simulink model "EV6_LUT_FourWheel_EV6Battery77p4kWh_PowerCorrected"  (R2024a)
settings: Solver=ode4  StartTime=0  StopTime=60  FixedStep=0.001  RelTol=1e-3
PreLoadFcn:
  | VSS_BICYCLE=Simulink.Variant('Dual=0');
  | VSS_DUAL=Simulink.Variant('Dual=1');
  | Dual=1;
  | load('DriveCycle2.mat')
PostLoadFcn:
  | if any(exist('dsrtsu_mdlpostloadfcn', 'file') ~= 0), dsrtsu_mdlpostloadfcn('Execute', bdroot); end
InitFcn:
  | , if any(exist('rtifpga_mdlclblib', 'file') ~= 0), rtifpga_mdlclblib('Init', bdroot); end,
  | , if any(exist('dsmpb_private', 'file') ~= 0), dsmpb_private('dsmpb_mdlclblib', 'Init', bdroot); end,
  | load('DriveCycle2.mat')
model workspace (MAT data in the model file):
  DiffRatio = 10.65
  EV6_2023_BattBranchCapacity_Ah = 55.5236728838
  EV6_2023_BattEnergy_kWh = 77.4
  EV6_2023_BattNominalVoltage_V = 697
  EV6_2023_BattNumCellsParallel = 2
  EV6_2023_BattNumCellsSeries = 192
  EV6_2023_BattOpenVoltCapBpts = [0 0.1 0.2 0.3 0.4 0.5 0.6 0.7 0.8 0.9 1]
  EV6_2023_BattOpenVoltTbl = [2.96762142548 3.40364281191 3.47417488548 3.54470541822 3.61523441014 3.68576186124 3.75628777151 3.82681214095 3.94527005036 4.07101207308 4.2120755254]
  EV6_2023_BattPackCapacity_Ah = 111.047345768
  EV6_2023_BattResistSocBpts = [0 0.2 0.4 0.6 0.8 1]
  EV6_2023_BattResistTbl = [0.0163620057716 0.0118174152018 0.00807187352333 0.00375663957972 0.00266904525531 0.00103635901355 0.0019014404175 0.0172368903217 0.0121226074867 0.00758541551769 0.00474065349228 0.00337561163613 ... (42 elements, 7x6)]
  EV6_2023_BattResistTempBpts = [243.1 253.1 263.1 273.1 283.1 298.1 313.1]
  EV6_2023_InitialPackOCV_V = 726.471714233
  EV6_2023_InitialSOC = 0.638878863672
  EV6_BattCellCapacity_Ah = 60.3
  EV6_BattInitialSOC = 0.638878863672
  EV6_BattOCV_Cell_V = [2.96762142548 3.40364281191 3.47417488548 3.54470541822 3.61523441014 3.68576186124 3.75628777151 3.82681214095 3.94527005036 4.07101207308 4.2120755254]
  EV6_BattOCV_SOC = [0 0.1 0.2 0.3 0.4 0.5 0.6 0.7 0.8 0.9 1]
  EV6_BattPackCapacity_Ah = 120.6
  EV6_BattParallelCells = 2
  EV6_BattResistanceSOC = [0 0.2 0.4 0.6 0.8 1]
  EV6_BattResistanceTable_Ohm = [0.0163620057716 0.0118174152018 0.00807187352333 0.00375663957972 0.00266904525531 0.00103635901355 0.0019014404175 0.0172368903217 0.0121226074867 0.00758541551769 0.00474065349228 0.00337561163613 ... (42 elements, 7x6)]
  EV6_BattResistanceTemp_K = [243.1 253.1 263.1 273.1 283.1 298.1 313.1]
  EV6_BattSeriesCells = 192
  EV6_FinalDriveRatio = 10.65
  EV6_TargetPackResistance_Ohm = 0.132763804608
  Gas = 0.383333333333
undefined symbols (not defined in the file): accel_bp_mps2, AccelCmd, ActTqLF_Nm_, ActTqLR_Nm_, ActTqRF_Nm_, ActTqRR_Nm_, BattChargeLimitMaxPwr, BattChargeLimitSocBpts, BattChargeLimitTbl, BattDischargeLimitSocBpts, BattDischargeLimitTbl, BattDischargeMaxPwr, BrakeMaxPrs, BrakeMaxTrq, ChassisDistCg2FrontAxle, ChassisDistCg2RearAxle, ChassisVehMass, CltchCmd, CoastDown, DecelCmd, DiscIntNeverNeededParam, EnvGravCnst, EnvPrs, EnvTemp, EV6_RegenTorqueGain, EV6_TractionTorqueGain, front_share_regen_3d, front_share_traction_3d, FuelSpecificGrav, GearCmd, h, InitStates, lgSw, limitedMCT, MCT, MtrEffSpdBpts, MtrEffTbl, MtrEffTrqBpts, MtrPwrMax, MtrTrqMax, out_1, pMCT, RealSimPara, Ref_speed, Ref_time, regen_torque_bp_Nm, speed_bp_kph, SteeringCmd, SupvsryCtrlRegenBrkCutOffTbl, SupvsryCtrlRegenSpdBpts, TestScnrioCycleNum, traction_torque_bp_Nm, US06, VEH
libraries: VSIGenLib x65, simulink x54, etargetslib x38, dsmpblib x24, vehdynlibtire x12, autolibshared x11, vehdynlibsuspension x7, vehdynlibtirecommon x7, autolibpowerinfoutils x6, autolibutils x5, autolibsharedcoupling x4, autolibmappedmotor x4
(part 8 of 19)

== system EV6_LUT_FourWheel_EV6Battery77p4kWh_PowerCorrected/Vehicle Under Test1/Vehicle/Powertrain Supervisory Controller /Engine Torque Command/EV6 Torque Distribution ==
  Accel_mps2 : Inport
  Speed_kph : Inport  Port=2
  MtrTrqCmd : Inport  Port=3
  Regen Brake Split LUT : Subsystem
  Select Front Share : Switch  SaturateOnIntegerOverflow=off  InputSameDT=off
  Select Front Torque : Switch  SaturateOnIntegerOverflow=off  InputSameDT=off
  Select Rear Share : Switch  SaturateOnIntegerOverflow=off  InputSameDT=off
  Select Rear Torque : Switch  SaturateOnIntegerOverflow=off  InputSameDT=off
  Share Sum : Sum
  Share Sum Display : Display
  Torque Error : Sum  Inputs=+-
  Torque Error Display : Display
  Torque Sum : Sum
  Traction Torque Split LUT : Subsystem
  FrontShare : Outport
  RearShare : Outport  Port=2
  FrontMtrTrqCmd : Outport  Port=3
  RearMtrTrqCmd : Outport  Port=4
  wires:
  Accel_mps2/1 -> Traction Torque Split LUT/1(Accel_mps2), Regen Brake Split LUT/1(Accel_mps2)
  Speed_kph/1 -> Traction Torque Split LUT/2(Speed_kph), Regen Brake Split LUT/2(Speed_kph)
  MtrTrqCmd/1 -> Select Rear Torque/2, Torque Error/2, Select Front Torque/2, Select Front Share/2, Select Rear Share/2, Traction Torque Split LUT/3(MtrTrqCmd), Regen Brake Split LUT/3(MtrTrqCmd)
  Traction Torque Split LUT/1(FrontShare) -> Select Front Share/1
  Regen Brake Split LUT/1(FrontShare) -> Select Front Share/3
  Traction Torque Split LUT/2(RearShare) -> Select Rear Share/1
  Regen Brake Split LUT/2(RearShare) -> Select Rear Share/3
  Traction Torque Split LUT/3(FrontMtrTrqCmd) -> Select Front Torque/1
  Regen Brake Split LUT/3(FrontMtrTrqCmd) -> Select Front Torque/3
  Traction Torque Split LUT/4(RearMtrTrqCmd) -> Select Rear Torque/1
  Regen Brake Split LUT/4(RearMtrTrqCmd) -> Select Rear Torque/3
  Select Front Share/1 -> FrontShare/1, Share Sum/1
  Select Rear Share/1 -> RearShare/1, Share Sum/2
  Select Front Torque/1 -> FrontMtrTrqCmd/1, Torque Sum/1
  Select Rear Torque/1 -> RearMtrTrqCmd/1, Torque Sum/2
  Share Sum/1 -> Share Sum Display/1
  Torque Sum/1 -> Torque Error/1
  Torque Error/1 -> Torque Error Display/1

== system EV6_LUT_FourWheel_EV6Battery77p4kWh_PowerCorrected/Vehicle Under Test1/Vehicle/Powertrain Supervisory Controller /Engine Torque Command/Motor Torque Arbitration and Power Management ==
  MotTrqCmdTrac : Inport
  AccelPdl : Inport  Port=2
  BattPwrDisChrgLmt : Inport  Port=3
  "BattPwrChrgLmt " : Inport  Port=4
  MotSpd : Inport  Port=5
  MotTrqCmdRegen : Inport  Port=6
  Accel Decel Switch : Switch  Criteria=u2 > Threshold  SaturateOnIntegerOverflow=off  InputSameDT=off
  Compare To Constant : simulink/Logic and Bit Operations/Compare To Constant  relop=>  const=0  OutDataTypeStr=boolean
  Power Management : Subsystem
  MotTrqCmdFinal : Outport  VectorParamsAs1DForOutWhenUnconnected=off
  wires:
  AccelPdl/1 -> Compare To Constant/1
  MotTrqCmdRegen/1 -> Accel Decel Switch/3
  MotTrqCmdTrac/1 -> Accel Decel Switch/1
  Power Management/1(MotTrqCmdFinal) -> MotTrqCmdFinal/1
  Accel Decel Switch/1 -> Power Management/4(MotTrqCmd)
  BattPwrDisChrgLmt/1 -> Power Management/1(BattPwrDischrgLmt)
  "BattPwrChrgLmt "/1 -> Power Management/2(BattPwrChrgLmt)
  MotSpd/1 -> Power Management/3(MotSpd)
  Compare To Constant/1 -> Accel Decel Switch/2

== system EV6_LUT_FourWheel_EV6Battery77p4kWh_PowerCorrected/Vehicle Under Test1/Vehicle/Powertrain Supervisory Controller /Engine Torque Command/Series Regen Braking ==
  note: - Total brake torque request based on brake pressure and parameters of disc brakes
      | - Use as much regenerative motor braking as possible
      | - Any braking torque request that cannot be provided by the motor, will be provided by the friction brakes
  note: These are all torque on wheels, which is DiffRatio*torque on motor
  BattSoc : Inport
  VehSpd : Inport  Port=2
  MotSpd : Inport  Port=3
  "DecelCmd " : Inport  Port=4
  BrkTrqReqTotal Display : Display
  ChrgLmt : Lookup_n-D  NumberOfTableDimensions=1  BreakpointsForDimension1=BattChargeLimitSocBpts  Table=BattChargeLimitTbl  ExtrapMethod=Clip  UseLastTableValue=on  InternalRulePriority=Speed  RndMeth=Simplest
  ChrgLmt Display : Display
  DecelCmd input : Display
  Display : Display
  Gain : Gain  Gain=-1
  Gain1 : Gain  Gain=BrakeMaxTrq
  Gain2 : Gain  Gain=1/BrakeMaxTrq
  Gain3 : Gain  Gain=EV6_FinalDriveRatio
  Max Motor Torque : LibPtSupervisoryCtrl/Powertrain Supervisory Controller /Engine Torque Command/Accel Pedal to Traction Wheel Torque Request/Max Motor Torque  SystemSampleTime=-1  VariantActivationTime=update diagram  AllowFlexibleInterface=on  Latency=0  AutoFrameSizeCalculation=off
  MinMax : MinMax  Inputs=2
  MotSpd Display : Display
  MotTrqCmdRegen : Display
  MotTrqReflectedToWheels1 : Gain  Commented=on  Gain=DiffRatio
  Product1 : Product
  Product3 : Product
  RegenBraking Display : Display
  RegenBrakingCutoff : Lookup_n-D  NumberOfTableDimensions=1  BreakpointsForDimension1=SupvsryCtrlRegenSpdBpts  Table=SupvsryCtrlRegenBrkCutOffTbl  ExtrapMethod=Clip  UseLastTableValue=on  InternalRulePriority=Speed  RndMeth=Simplest
  RegenFactor Display : Display
  Saturation : Saturate  UpperLimit=1  LowerLimit=0
  Saturation1 : Saturate  UpperLimit=1  LowerLimit=0
  Scope{,1..6} (7 alike) : Scope
  Subtract : Sum  Inputs=+-
  VehSpd Display : Display
  WhlTrqReflectedToMot : Gain  Gain=1/EV6_FinalDriveRatio
  WhlTrqReflectedToMot1 : Gain  Commented=on  Gain=1/DiffRatio
  " MotTrqCmdRegen" : Outport  VectorParamsAs1DForOutWhenUnconnected=off
  " BrkCmd" : Outport  Port=2  VectorParamsAs1DForOutWhenUnconnected=off
  wires:
  Gain1/1 -> Scope/1, Subtract/1, MinMax/1  "BrkTrqReqTotal"
  Product3/1 -> WhlTrqReflectedToMot/1, Subtract/2  "MotTrqRegenWhl"
  Saturation1/1 -> Scope3/1, " BrkCmd"/1
  Max Motor Torque/1 -> Gain3/1, Scope6/1  "MotTrqMax"
  MinMax/1 -> Product3/1  "min"
  ChrgLmt/1 -> ChrgLmt Display/1, Product1/2
  VehSpd/1 -> VehSpd Display/1, RegenBrakingCutoff/1
  RegenBrakingCutoff/1 -> RegenBraking Display/1, Product1/1
  Product1/1 -> RegenFactor Display/1, Scope5/1, Product3/2  "RegenFactor"
  BattSoc/1 -> ChrgLmt/1
  MotSpd/1 -> MotSpd Display/1, Max Motor Torque/1
  Gain3/1 -> Scope1/1, MinMax/2  "MotTrqMaxWhls"
  WhlTrqReflectedToMot/1 -> Gain/1
  Gain/1 -> MotTrqCmdRegen/1, Scope4/1, " MotTrqCmdRegen"/1  "MotTrqCmdRegen"
  "DecelCmd "/1 -> Saturation/1, DecelCmd input/1  "BrkPrsReq"
  Saturation/1 -> Display/1, Scope2/1, Gain1/1
  Subtract/1 -> Gain2/1
  Gain2/1 -> BrkTrqReqTotal Display/1, Saturation1/1  "BrkTrqReqTotal"

== system EV6_LUT_FourWheel_EV6Battery77p4kWh_PowerCorrected/Vehicle Under Test1/Vehicle/Rear Wheel Drive/Ideal Diff/Power Bus ==
  DriveshftTrq : Inport
  Speed : Inport  Port=2
  Bus Creator : BusCreator  Inputs=1
  Bus Creator5 : BusCreator  Inputs=2
  Bus Creator6 : BusCreator  Inputs=3
  Bus Creator7 : BusCreator  Inputs=1
  Constant : Constant  Value=0
  Constant1 : Constant  Value=0
  Constant2 : Constant  Value=0
  Demux : Demux  Outputs=3
  Power Accounting Bus Creator : autolibpowerinfoutils/Power Accounting Bus Creator  AssctBlkSelPopup=Parent reference block  RefBlkName='autolibshareddiff/Open Differential'  PwrTrnsfrdCheckBox=on  PwrNotTrnsfrdCheckBox=on  PwrStoredCheckBox=on  aMode=aMode
  Signal Specification5 : SignalSpecification  Unit=W
  Transferred Power : Product
  Vector Concatenate : Concatenate  NumInputs=3
  PwrInfo : Outport
  wires:
  Constant2/1 -> Bus Creator7/1  "PwrStoredShft"
  Constant1/1 -> Bus Creator5/2  "PwrDampLoss"
  Vector Concatenate/1 -> Demux/1
  Speed/1 -> Transferred Power/2
  Demux/1 -> Bus Creator6/1  "PwrDriveshft"
  Demux/2 -> Bus Creator6/2  "PwrAxl1"
  Bus Creator7/1 -> Power Accounting Bus Creator/3
  DriveshftTrq/1 -> Transferred Power/1
  Demux/3 -> Bus Creator6/3  "PwrAxl2"
  Constant/1 -> Bus Creator5/1  "PwrMechLoss"
  Signal Specification5/1 -> Vector Concatenate/1, Vector Concatenate/2, Vector Concatenate/3  "PwrDriveshft"
  Transferred Power/1 -> Signal Specification5/1
  Bus Creator6/1 -> Bus Creator/1  "PwrTrnsfrd"
  Bus Creator5/1 -> Power Accounting Bus Creator/2
  Power Accounting Bus Creator/1 -> PwrInfo/1  "PwrInfo"
  Bus Creator/1 -> Power Accounting Bus Creator/1

== system EV6_LUT_FourWheel_EV6Battery77p4kWh_PowerCorrected/Vehicle Under Test1/Vehicle/Rear Wheel Drive/Ideal Diff AWD/Power Bus ==
  DriveshftTrq : Inport
  Speed : Inport  Port=2
  Bus Creator : BusCreator  Inputs=1
  Bus Creator5 : BusCreator  Inputs=2
  Bus Creator6 : BusCreator  Inputs=3
  Bus Creator7 : BusCreator  Inputs=1
  Constant : Constant  Value=0
  Constant1 : Constant  Value=0
  Constant2 : Constant  Value=0
  Demux : Demux  Outputs=3
  Power Accounting Bus Creator : autolibpowerinfoutils/Power Accounting Bus Creator  AssctBlkSelPopup=Parent reference block  RefBlkName='autolibshareddiff/Open Differential'  PwrTrnsfrdCheckBox=on  PwrNotTrnsfrdCheckBox=on  PwrStoredCheckBox=on  aMode=aMode
  Signal Specification5 : SignalSpecification  Unit=W
  Transferred Power : Product
  Vector Concatenate : Concatenate  NumInputs=3
  PwrInfo : Outport
  wires:
  Constant2/1 -> Bus Creator7/1  "PwrStoredShft"
  Constant1/1 -> Bus Creator5/2  "PwrDampLoss"
  Vector Concatenate/1 -> Demux/1
  Speed/1 -> Transferred Power/2
  Demux/1 -> Bus Creator6/1  "PwrDriveshft"
  Demux/2 -> Bus Creator6/2  "PwrAxl1"
  Bus Creator7/1 -> Power Accounting Bus Creator/3
  DriveshftTrq/1 -> Transferred Power/1
  Demux/3 -> Bus Creator6/3  "PwrAxl2"
  Constant/1 -> Bus Creator5/1  "PwrMechLoss"
  Signal Specification5/1 -> Vector Concatenate/1, Vector Concatenate/2, Vector Concatenate/3  "PwrDriveshft"
  Transferred Power/1 -> Signal Specification5/1
  Bus Creator6/1 -> Bus Creator/1  "PwrTrnsfrd"
  Bus Creator5/1 -> Power Accounting Bus Creator/2
  Power Accounting Bus Creator/1 -> PwrInfo/1  "PwrInfo"
  Bus Creator/1 -> Power Accounting Bus Creator/1

== system EV6_LUT_FourWheel_EV6Battery77p4kWh_PowerCorrected/Vehicle Under Test1/Vehicle/Rear Wheel Drive/Real Diff/Power Bus ==
  DriveshftTrq : Inport
  Speed : Inport  Port=2
  Bus Creator : BusCreator  Inputs=1
  Bus Creator5 : BusCreator  Inputs=2
  Bus Creator6 : BusCreator  Inputs=3
  Bus Creator7 : BusCreator  Inputs=1
  Constant : Constant  Value=0
  Constant1 : Constant  Value=0
  Constant2 : Constant  Value=0
  Demux : Demux  Outputs=3
  Power Accounting Bus Creator : autolibpowerinfoutils/Power Accounting Bus Creator  AssctBlkSelPopup=Parent reference block  RefBlkName='autolibshareddiff/Open Differential'  PwrTrnsfrdCheckBox=on  PwrNotTrnsfrdCheckBox=on  PwrStoredCheckBox=on  aMode=aMode
  Signal Specification5 : SignalSpecification  Unit=W
  Transferred Power : Product
  Vector Concatenate : Concatenate  NumInputs=3
  PwrInfo : Outport
  wires:
  Constant2/1 -> Bus Creator7/1  "PwrStoredShft"
  Constant1/1 -> Bus Creator5/2  "PwrDampLoss"
  Vector Concatenate/1 -> Demux/1
  Speed/1 -> Transferred Power/2
  Demux/1 -> Bus Creator6/1  "PwrDriveshft"
  Demux/2 -> Bus Creator6/2  "PwrAxl1"
  Bus Creator7/1 -> Power Accounting Bus Creator/3
  DriveshftTrq/1 -> Transferred Power/1
  Demux/3 -> Bus Creator6/3  "PwrAxl2"
  Constant/1 -> Bus Creator5/1  "PwrMechLoss"
  Signal Specification5/1 -> Vector Concatenate/1, Vector Concatenate/2, Vector Concatenate/3  "PwrDriveshft"
  Transferred Power/1 -> Signal Specification5/1
  Bus Creator6/1 -> Bus Creator/1  "PwrTrnsfrd"
  Bus Creator5/1 -> Power Accounting Bus Creator/2
  Power Accounting Bus Creator/1 -> PwrInfo/1  "PwrInfo"
  Bus Creator/1 -> Power Accounting Bus Creator/1

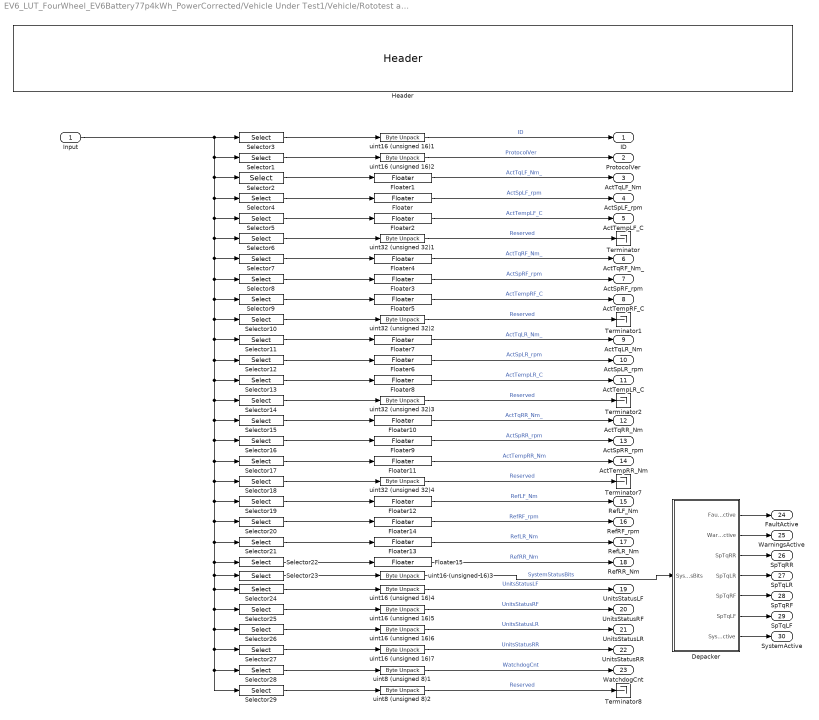
== system EV6_LUT_FourWheel_EV6Battery77p4kWh_PowerCorrected/Vehicle Under Test1/Vehicle/Rototest and ORNL Interface/From Rototest/RotoTestEthRX ==
  Input : Inport
  Depacker : Subsystem
  Floater{,1..15} (16 alike) : VSIGenLib/Floater  SystemSampleTime=-1  VariantActivationTime=update diagram  AllowFlexibleInterface=on  Latency=0  AutoFrameSizeCalculation=off
  Header : VSIGenLib/Header  not=''
  Selector1 : Selector  IndexMode=Zero-based  InputPortWidth=96  IndexOptions=Index vector (dialog)  Indices=[3 2]  OutputSizes=1
  Selector10 : Selector  IndexMode=Zero-based  InputPortWidth=96  IndexOptions=Index vector (dialog)  Indices=[35 34 33 32]  OutputSizes=1
  Selector11 : Selector  IndexMode=Zero-based  InputPortWidth=96  IndexOptions=Index vector (dialog)  Indices=[39 38 37 36]  OutputSizes=1
  Selector12 : Selector  IndexMode=Zero-based  InputPortWidth=96  IndexOptions=Index vector (dialog)  Indices=[43 42 41 40]  OutputSizes=1
  Selector13 : Selector  IndexMode=Zero-based  InputPortWidth=96  IndexOptions=Index vector (dialog)  Indices=[47 46 45 44]  OutputSizes=1
  Selector14 : Selector  IndexMode=Zero-based  InputPortWidth=96  IndexOptions=Index vector (dialog)  Indices=[51 50 49 48]  OutputSizes=1
  Selector15 : Selector  IndexMode=Zero-based  InputPortWidth=96  IndexOptions=Index vector (dialog)  Indices=[55 54 53 52]  OutputSizes=1
  Selector16 : Selector  IndexMode=Zero-based  InputPortWidth=96  IndexOptions=Index vector (dialog)  Indices=[59 58 57 56]  OutputSizes=1
  Selector17 : Selector  IndexMode=Zero-based  InputPortWidth=96  IndexOptions=Index vector (dialog)  Indices=[63 62 61 60]  OutputSizes=1
  Selector18 : Selector  IndexMode=Zero-based  InputPortWidth=96  IndexOptions=Index vector (dialog)  Indices=[67 66 65 64]  OutputSizes=1
  Selector19 : Selector  IndexMode=Zero-based  InputPortWidth=96  IndexOptions=Index vector (dialog)  Indices=[71 70 69 68]  OutputSizes=1
  Selector2 : Selector  IndexMode=Zero-based  InputPortWidth=96  IndexOptions=Index vector (dialog)  Indices=[7 6 5 4]  OutputSizes=1
  Selector20 : Selector  IndexMode=Zero-based  InputPortWidth=96  IndexOptions=Index vector (dialog)  Indices=[75 74 73 72]  OutputSizes=1
  Selector21 : Selector  IndexMode=Zero-based  InputPortWidth=96  IndexOptions=Index vector (dialog)  Indices=[79 78 77 76]  OutputSizes=1
  Selector22 : Selector  IndexMode=Zero-based  InputPortWidth=96  IndexOptions=Index vector (dialog)  Indices=[83 82 81 80]  OutputSizes=1
  Selector23 : Selector  IndexMode=Zero-based  InputPortWidth=96  IndexOptions=Index vector (dialog)  Indices=[85 84]  OutputSizes=1
  Selector24 : Selector  IndexMode=Zero-based  InputPortWidth=96  IndexOptions=Index vector (dialog)  Indices=[87 86]  OutputSizes=1
  Selector25 : Selector  IndexMode=Zero-based  InputPortWidth=96  IndexOptions=Index vector (dialog)  Indices=[89 88]  OutputSizes=1
  Selector26 : Selector  IndexMode=Zero-based  InputPortWidth=96  IndexOptions=Index vector (dialog)  Indices=[91 90]  OutputSizes=1
  Selector27 : Selector  IndexMode=Zero-based  InputPortWidth=96  IndexOptions=Index vector (dialog)  Indices=[93 92]  OutputSizes=1
  Selector28 : Selector  IndexMode=Zero-based  InputPortWidth=96  IndexOptions=Index vector (dialog)  Indices=[94]  OutputSizes=1
  Selector29 : Selector  IndexMode=Zero-based  InputPortWidth=96  IndexOptions=Index vector (dialog)  Indices=[95]  OutputSizes=1
  Selector3 : Selector  IndexMode=Zero-based  InputPortWidth=96  IndexOptions=Index vector (dialog)  Indices=[1 0]  OutputSizes=1
  Selector4 : Selector  IndexMode=Zero-based  InputPortWidth=96  IndexOptions=Index vector (dialog)  Indices=[11 10 9 8]  OutputSizes=1
  Selector5 : Selector  IndexMode=Zero-based  InputPortWidth=96  IndexOptions=Index vector (dialog)  Indices=[15 14 13 12]  OutputSizes=1
  Selector6 : Selector  IndexMode=Zero-based  InputPortWidth=96  IndexOptions=Index vector (dialog)  Indices=[19 18 17 16]  OutputSizes=1
  Selector7 : Selector  IndexMode=Zero-based  InputPortWidth=96  IndexOptions=Index vector (dialog)  Indices=[23 22 21 20]  OutputSizes=1
  Selector8 : Selector  IndexMode=Zero-based  InputPortWidth=96  IndexOptions=Index vector (dialog)  Indices=[27 26 25 24]  OutputSizes=1
  Selector9 : Selector  IndexMode=Zero-based  InputPortWidth=96  IndexOptions=Index vector (dialog)  Indices=[31 30 29 28]  OutputSizes=1
  Terminator{,1..2,7..8} (5 alike) : Terminator
  uint16 (unsigned 16){1..7} (7 alike) : etargetslib/Byte Unpack  dimensions={[1]}  datatypes={'uint16'}  byteAlign=1
  uint32 (unsigned 32){1..4} (4 alike) : etargetslib/Byte Unpack  dimensions={[1]}  datatypes={'uint32'}  byteAlign=1
  uint8 (unsigned 8)1 : etargetslib/Byte Unpack  dimensions={[1]}  datatypes={'uint8'}  byteAlign=1
  uint8 (unsigned 8)2 : etargetslib/Byte Unpack  dimensions={[1]}  datatypes={'uint8'}  byteAlign=1
  ID : Outport
  ProtocolVer : Outport  Port=2
  ActTqLF_Nm : Outport  Port=3
  ActSpLF_rpm : Outport  Port=4
  ActTempLF_C : Outport  Port=5
  ActTqRF_Nm_ : Outport  Port=6
  ActSpRF_rpm : Outport  Port=7
  ActTempRF_C : Outport  Port=8
  ActTqLR_Nm : Outport  Port=9
  ActSpLR_rpm : Outport  Port=10
  ActTempLR_C : Outport  Port=11
  ActTqRR_Nm : Outport  Port=12
  ActSpRR_rpm : Outport  Port=13
  ActTempRR_Nm : Outport  Port=14
  RefLF_Nm : Outport  Port=15
  RefRF_rpm : Outport  Port=16
  RefLR_Nm : Outport  Port=17
  RefRR_Nm : Outport  Port=18
  UnitsStatusLF : Outport  Port=19
  UnitsStatusRF : Outport  Port=20
  UnitsStatusLR : Outport  Port=21
  UnitsStatusRR : Outport  Port=22
  WatchdogCnt : Outport  Port=23
  FaultActive : Outport  Port=24
  WarningsActive : Outport  Port=25
  SpTqRR : Outport  Port=26
  SpTqLR : Outport  Port=27
  SpTqRF : Outport  Port=28
  SpTqLF : Outport  Port=29
  SystemActive : Outport  Port=30
  wires:
  Selector11/1 -> Floater7/1
  Floater10/1 -> ActTqRR_Nm/1  "ActTqRR_Nm_"
  Selector4/1 -> Floater/1
  Selector1/1 -> uint16 (unsigned 16)2/1
  Selector10/1 -> uint32 (unsigned 32)2/1
  Selector19/1 -> Floater12/1
  Input/1 -> Selector3/1, Selector1/1, Selector2/1, Selector4/1, Selector5/1, Selector6/1, Selector14/1, Selector15/1, Selector16/1, Selector24/1, Selector28/1, Selector29/1, Selector27/1, Selector26/1, Selector25/1, Selector23/1, Selector22/1, Selector21/1, Selector20/1, Selector19/1, Selector18/1, Selector17/1, Selector13/1, Selector12/1, Selector11/1, Selector10/1, Selector9/1, Selector8/1, Selector7/1
  Selector21/1 -> Floater13/1
  Selector29/1 -> uint8 (unsigned 8)2/1
  Selector28/1 -> uint8 (unsigned 8)1/1
  Selector3/1 -> uint16 (unsigned 16)1/1
  Floater8/1 -> ActTempLR_C/1  "ActTempLR_C"
  Selector16/1 -> Floater9/1
  Selector15/1 -> Floater10/1
  Selector5/1 -> Floater2/1
  Selector9/1 -> Floater5/1
  Selector20/1 -> Floater14/1
  Floater6/1 -> ActSpLR_rpm/1  "ActSpLR_rpm"
  Floater11/1 -> ActTempRR_Nm/1  "ActTempRR_Nm"
  uint8 (unsigned 8)2/1 -> Terminator8/1  "Reserved"
  Floater4/1 -> ActTqRF_Nm_/1  "ActTqRF_Nm_"
  Selector25/1 -> uint16 (unsigned 16)5/1
  Floater3/1 -> ActSpRF_rpm/1  "ActSpRF_rpm"
  uint32 (unsigned 32)4/1 -> Terminator7/1  "Reserved"
  uint16 (unsigned 16)3/1 -> Depacker/1(SysStsBits)  "SystemStatusBits"
  Selector6/1 -> uint32 (unsigned 32)1/1
  Selector26/1 -> uint16 (unsigned 16)6/1
  Selector13/1 -> Floater8/1
  Selector2/1 -> Floater1/1
  Selector14/1 -> uint32 (unsigned 32)3/1
  Floater13/1 -> RefLR_Nm/1  "RefLR_Nm"
  Selector27/1 -> uint16 (unsigned 16)7/1
  uint16 (unsigned 16)4/1 -> UnitsStatusLF/1  "UnitsStatusLF"
  Selector17/1 -> Floater11/1
  uint16 (unsigned 16)6/1 -> UnitsStatusLR/1  "UnitsStatusLR"
  Selector23/1 -> uint16 (unsigned 16)3/1
  Selector12/1 -> Floater6/1
  Selector18/1 -> uint32 (unsigned 32)4/1
  Selector22/1 -> Floater15/1
  uint16 (unsigned 16)7/1 -> UnitsStatusRR/1  "UnitsStatusRR"
  Selector8/1 -> Floater3/1
  Selector7/1 -> Floater4/1
  Selector24/1 -> uint16 (unsigned 16)4/1
  uint16 (unsigned 16)2/1 -> ProtocolVer/1  "ProtocolVer"
  Floater7/1 -> ActTqLR_Nm/1  "ActTqLR_Nm_"
  Floater12/1 -> RefLF_Nm/1  "RefLF_Nm"
  Floater2/1 -> ActTempLF_C/1  "ActTempLF_C"
  Floater1/1 -> ActTqLF_Nm/1  "ActTqLF_Nm_"
  Floater9/1 -> ActSpRR_rpm/1  "ActSpRR_rpm"
  uint32 (unsigned 32)3/1 -> Terminator2/1  "Reserved"
  uint16 (unsigned 16)5/1 -> UnitsStatusRF/1  "UnitsStatusRF"
  Floater14/1 -> RefRF_rpm/1  "RefRF_rpm"
  uint8 (unsigned 8)1/1 -> WatchdogCnt/1  "WatchdogCnt"
  Floater15/1 -> RefRR_Nm/1  "RefRR_Nm"
  uint16 (unsigned 16)1/1 -> ID/1  "ID"
  uint32 (unsigned 32)1/1 -> Terminator/1  "Reserved"
  Floater/1 -> ActSpLF_rpm/1  "ActSpLF_rpm"
  uint32 (unsigned 32)2/1 -> Terminator1/1  "Reserved"
  Floater5/1 -> ActTempRF_C/1  "ActTempRF_C"
  Depacker/6(SpTqLF) -> SpTqLF/1
  Depacker/4(SpTqLR) -> SpTqLR/1
  Depacker/3(SpTqRR) -> SpTqRR/1
  Depacker/2(WarningsActive) -> WarningsActive/1
  Depacker/1(FaultActive) -> FaultActive/1
  Depacker/5(SpTqRF) -> SpTqRF/1
  Depacker/7(SystemActive) -> SystemActive/1

== system EV6_LUT_FourWheel_EV6Battery77p4kWh_PowerCorrected/Vehicle Under Test1/Vehicle/Rototest and ORNL Interface/Get Wheel Spd Cmd Based on Wheel Dynamics/WheelSpdCmd ==
  In1 : Inport
  Bus Selector : BusSelector  OutputSignals=PT IF WFL rotv,PT IF WFR rotv,PT IF WRL rotv,PT IF WRR rotv
  Mux : Mux
  Out1 : Outport
  wires:
  Bus Selector/2 -> Mux/2  "<PT IF WFR rotv>"
  Bus Selector/3 -> Mux/3  "<PT IF WRL rotv>"
  In1/1 -> Bus Selector/1
  Bus Selector/4 -> Mux/4  "<PT IF WRR rotv>"
  Bus Selector/1 -> Mux/1  "<PT IF WFL rotv>"
  Mux/1 -> Out1/1

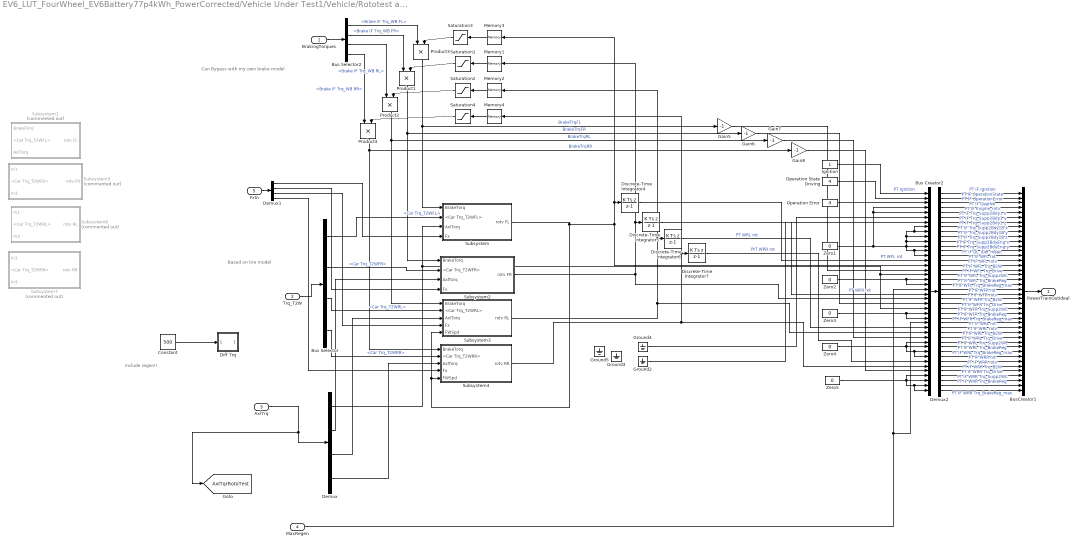
== system EV6_LUT_FourWheel_EV6Battery77p4kWh_PowerCorrected/Vehicle Under Test1/Vehicle/Rototest and ORNL Interface/Get Wheel Spd Cmd Based on Wheel Dynamics/Whl Dynamics & Format CM Powertrain Signal ==
  note: Can Bypass with my own brake model
  note: Based on tire model
  note: include regen!!
  BrakingTorques : Inport
  Trq_T2W : Inport  Port=2
  AxlTrq : Inport  Port=3
  MaxRegen : Inport  Port=4
  FxIn : Inport  Port=5
  Bus Creator2 : BusCreator  Inputs=42
  Bus Selector : BusSelector  OutputSignals=Car Trq_T2WFL,Car Trq_T2WFR,Car Trq_T2WRL,Car Trq_T2WRR
  Bus Selector2 : BusSelector  OutputSignals=Brake IF Trq_WB FL,Brake IF Trq_WB FR,Brake IF Trq_WB RL,Brake IF Trq_WB RR
  BusCreator1 : BusCreator  Inputs=42
  Constant : Constant  Value=500
  Demux : Demux
  Demux1 : Demux
  Demux2 : Demux  Outputs=42
      settings: DisplayOption=none
  Diff Trq : Subsystem
  Discrete-Time Integrator{4..7} (4 alike) : DiscreteIntegrator  IntegratorMethod=Integration: Backward Euler  SampleTime=-1  ICPrevOutput=DiscIntNeverNeededParam  ICPrevScaledInput=DiscIntNeverNeededParam
  Gain{5..8} (4 alike) : Gain  Gain=-1
  Ground{2..5} (4 alike) : Ground
  Ignition : Constant
  Memory{1..4} (4 alike) : Memory
  Operation Error : Constant  Value=4
  Operation State Driving : Constant  Value=4
  Product{1..4} (4 alike) : Product  RndMeth=Zero
  Saturation{1..4} (4 alike) : Saturate  UpperLimit=1  LowerLimit=-1
  Subsystem : Subsystem
  Subsystem1 : Subsystem  Commented=on
  Subsystem2 : Subsystem
  Subsystem3 : Subsystem
  Subsystem4 : Subsystem
  Subsystem5 : Subsystem  Commented=on
  Subsystem6 : Subsystem  Commented=on
  Subsystem7 : Subsystem  Commented=on
  Zero{1..5} (5 alike) : Constant  Value=0
  PowerTrainOutIdeal : Outport
  tag scope: AxlTqrRotoTest=global
  wires:
  Demux1/4 -> Subsystem4/4(Fx)
  Demux1/3 -> Subsystem3/4(Fx)
  Demux1/2 -> Subsystem2/4(Fx)
  Demux1/1 -> Subsystem/4(Fx)
  FxIn/1 -> Demux1/1
  Demux/4 -> Subsystem4/3(AxlTorq)
  Bus Selector/4 -> Subsystem4/2(<Car Trq_T2WRR>)  "<Car Trq_T2WRR>"
  Subsystem4/1(rotv RR) -> Bus Creator2/37, Discrete-Time Integrator7/1, Memory4/1
  Demux/3 -> Subsystem3/3(AxlTorq)
  Bus Selector/3 -> Subsystem3/2(<Car Trq_T2WRL>)  "<Car Trq_T2WRL>"
  Subsystem3/1(rotv RL) -> Bus Creator2/30, Discrete-Time Integrator6/1, Memory2/1
  Demux/2 -> Subsystem2/3(AxlTorq)
  Bus Selector/2 -> Subsystem2/2(<Car Trq_T2WFR>)  "<Car Trq_T2WFR>"
  Subsystem2/1(rotv FR) -> Discrete-Time Integrator5/1, Memory1/1, Bus Creator2/23
  Bus Selector/1 -> Subsystem/2(<Car Trq_T2WFL>)  "<Car Trq_T2WFL>"
  Subsystem/1(rotv FL) -> Discrete-Time Integrator4/1, Memory3/1, Bus Creator2/16, Subsystem4/5(FWSpd), Subsystem3/5(FWSpd)
  MaxRegen/1 -> Bus Creator2/21, Bus Creator2/28
  Demux/1 -> Bus Creator2/18, Bus Creator2/25, Subsystem/3(AxlTorq)
  AxlTrq/1 -> Demux/1, [AxlTqrRotoTest]
  Constant/1 -> Diff Trq/1(In1)
  Ground4/1 -> Bus Creator2/6
  Ground2/1 -> Bus Creator2/7
  BusCreator1/1 -> PowerTrainOutIdeal/1
  Demux2/1 -> BusCreator1/1  "PT IF Ignition"
  Demux2/2 -> BusCreator1/2  "PT IF OperationState"
  Demux2/3 -> BusCreator1/3  "PT IF OperationError"
  Demux2/4 -> BusCreator1/4  "PT IF GearNo"
  Demux2/5 -> BusCreator1/5  "PT IF Engine_rotv"
  Demux2/6 -> BusCreator1/6  "PT IF Trq_Supp2Bdy1 x"
  Demux2/7 -> BusCreator1/7  "PT IF Trq_Supp2Bdy1 y"
  Demux2/8 -> BusCreator1/8  "PT IF Trq_Supp2Bdy1 z"
  Demux2/9 -> BusCreator1/9  "PT IF Trq_Supp2Bdy1B x"
  Demux2/10 -> BusCreator1/10  "PT IF Trq_Supp2Bdy1B y"
  Demux2/11 -> BusCreator1/11  "PT IF Trq_Supp2Bdy1B z"
  Demux2/12 -> BusCreator1/12  "PT IF Trq_Supp2BdyEng x"
  Demux2/13 -> BusCreator1/13  "PT IF Trq_Supp2BdyEng y"
  Demux2/14 -> BusCreator1/14  "PT IF DL_iDiff_mean"
  Demux2/15 -> BusCreator1/15  "PT IF WFL rot"
  Demux2/16 -> BusCreator1/16  "PT IF WFL rotv"
  Demux2/17 -> BusCreator1/17  "PT IF WFL Trq_B2W"
  Demux2/18 -> BusCreator1/18  "PT IF WFL Trq_Drive"
  Demux2/19 -> BusCreator1/19  "PT IF WFL Trq_Supp2WC"
  Demux2/20 -> BusCreator1/20  "PT IF WFL Trq_BrakeReg"
  Demux2/21 -> BusCreator1/21  "PT IF WFL Trq_BrakeReg_max"
  Demux2/22 -> BusCreator1/22  "PT IF WFR rot"
  Demux2/23 -> BusCreator1/23  "PT IF WFR rotv"
  Demux2/24 -> BusCreator1/24  "PT IF WFR Trq_B2W"
  Demux2/25 -> BusCreator1/25  "PT IF WFR Trq_Drive"
  Demux2/26 -> BusCreator1/26  "PT IF WFR Trq_Supp2WC"
  Demux2/27 -> BusCreator1/27  "PT IF WFR Trq_BrakeReg"
  Demux2/28 -> BusCreator1/28  "PT IF WFR Trq_BrakeReg_max"
  Demux2/29 -> BusCreator1/29  "PT IF WRL rot"
  Demux2/30 -> BusCreator1/30  "PT IF WRL rotv"
  Demux2/31 -> BusCreator1/31  "PT IF WRL Trq_B2W"
  Demux2/32 -> BusCreator1/32  "PT IF WRL Trq_Drive"
  Demux2/33 -> BusCreator1/33  "PT IF WRL Trq_Supp2WC"
  Demux2/34 -> BusCreator1/34  "PT IF WRL Trq_BrakeReg"
  Demux2/35 -> BusCreator1/35  "PT IF WRL Trq_BrakeReg_max"
  Demux2/36 -> BusCreator1/36  "PT IF WRR rot"
  Demux2/37 -> BusCreator1/37  "PT IF WRR rotv"
  Demux2/38 -> BusCreator1/38  "PT IF WRR Trq_B2W"
  Demux2/39 -> BusCreator1/39  "PT IF WRR Trq_Drive"
  Demux2/40 -> BusCreator1/40  "PT IF WRR Trq_Supp2WC"
  Demux2/41 -> BusCreator1/41  "PT IF WRR Trq_BrakeReg"
  Demux2/42 -> BusCreator1/42  "PT IF WRR Trq_BrakeReg_max"
  Gain8/1 -> Bus Creator2/38
  Gain7/1 -> Bus Creator2/31
  Gain5/1 -> Bus Creator2/17
  Gain6/1 -> Bus Creator2/24
  Zero5/1 -> Bus Creator2/42, Bus Creator2/41, Bus Creator2/40, Bus Creator2/39
  Zero4/1 -> Bus Creator2/35, Bus Creator2/34, Bus Creator2/33, Bus Creator2/32
  Zero3/1 -> Bus Creator2/27, Bus Creator2/26
  Zero2/1 -> Bus Creator2/20, Bus Creator2/19
  Zero1/1 -> Bus Creator2/8, Bus Creator2/9, Bus Creator2/10, Bus Creator2/11, Bus Creator2/13, Bus Creator2/14, Bus Creator2/12, Bus Creator2/4, Bus Creator2/5
  Operation Error/1 -> Bus Creator2/3
  Operation State Driving/1 -> Bus Creator2/2
  Bus Creator2/1 -> Demux2/1
  Ignition/1 -> Bus Creator2/1  "PT Ignition"
  Discrete-Time Integrator4/1 -> Bus Creator2/15  "PT WFL rot"
  Discrete-Time Integrator5/1 -> Bus Creator2/22  "PT WFR rot"
  Discrete-Time Integrator6/1 -> Bus Creator2/29  "PT WRL rot"
  Discrete-Time Integrator7/1 -> Bus Creator2/36  "PtT WRR rot"
  Trq_T2W/1 -> Bus Selector/1
  BrakingTorques/1 -> Bus Selector2/1
  Product3/1 -> Gain5/1, Subsystem/1(BrakeTorq)  "BrakeTrqFL"
  Bus Selector2/1 -> Product3/1  "<Brake IF Trq_WB FL>"
  Saturation3/1 -> Product3/2
  Memory3/1 -> Saturation3/1
  Product1/1 -> Gain6/1, Subsystem2/1(BrakeTorq)  "BrakeTrqFR"
  Bus Selector2/2 -> Product1/1  "<Brake IF Trq_WB FR>"
  Memory1/1 -> Saturation1/1
  Saturation1/1 -> Product1/2
  Product2/1 -> Gain7/1, Subsystem3/1(BrakeTorq)  "BrakeTrqRL"
  Bus Selector2/3 -> Product2/1  "<Brake IF Trq_WB RL>"
  Memory2/1 -> Saturation2/1
  Saturation2/1 -> Product2/2
  Product4/1 -> Gain8/1, Subsystem4/1(BrakeTorq)  "BrakeTrqRR"
  Bus Selector2/4 -> Product4/1  "<Brake IF Trq_WB RR>"
  Memory4/1 -> Saturation4/1
  Saturation4/1 -> Product4/2

== system EV6_LUT_FourWheel_EV6Battery77p4kWh_PowerCorrected/Vehicle Under Test1/Vehicle/Rototest and ORNL Interface/To Rototest with Band-Aid/Band-Aid ==
  InSpd_rpm : Inport
  InTrq_Nm : Inport  Port=2
  BRAKE_PRESSED : Inport  Port=3
  VehSpd_kph : Inport  Port=4
  Band-Aid : Stateflow chart  TreatAsAtomicUnit=on
  BrkLatchThr_Nm : Constant  Value=-50
  Header : VSIGenLib/Header  not=''
  LaunchSpdThr_rpm : Constant  Value=2
  LaunchTrqThr_Nm : Constant  Value=20
  SettleTime_s : Constant  Value=5
  SpdLatchThr_rpm : Constant  Value=1e-5
  Terminator : Terminator
  Terminator1 : Terminator
  VehSpdThr_kph : Constant  Value=0.2
  dStop : Constant  Value=0
  OutMode : Outport
  OutSpd_rpm : Outport  Port=2
  tag scope: Mode=global
  wires:
  VehSpdThr_kph/1 -> Band-Aid/10(VehSpdThr_kph)
  VehSpd_kph/1 -> Band-Aid/9(VehSpd_kph)  "VehicleSpeed_kph"
  BRAKE_PRESSED/1 -> Band-Aid/4(BrkSw)
  dStop/1 -> Band-Aid/8(dStop)
  InTrq_Nm/1 -> Band-Aid/6(InTrq)  "InTrq_Nm"
  Band-Aid/2(OutSpd) -> OutSpd_rpm/1  "OutSpd"
  BrkLatchThr_Nm/1 -> Terminator1/1
  Band-Aid/1(OutMode) -> OutMode/1, [Mode]  "OutMode"
  SettleTime_s/1 -> Band-Aid/7(SettleTime)
  LaunchSpdThr_rpm/1 -> Band-Aid/1(LaunchSpdThr)
  Band-Aid/3(State) -> Terminator/1  "State"
  SpdLatchThr_rpm/1 -> Band-Aid/3(SpdLatchThr)
  LaunchTrqThr_Nm/1 -> Band-Aid/2(LaunchTrqThr)
  InSpd_rpm/1 -> Band-Aid/5(InSpd)  "InSpd_rpm"

== system EV6_LUT_FourWheel_EV6Battery77p4kWh_PowerCorrected/Vehicle Under Test1/Vehicle/Rototest and ORNL Interface/To Rototest with Band-Aid/Logging ==
  Ground1 : Ground
  RotoTestEthRXLogging : Subsystem
      mask Display:
      | color('white')
      | disp('RotTestEthLog')
      | port_label('output', 1, 'ID')
      | port_label('output', 2, 'ProtocolVer')
      | port_label('output', 3, 'ActTqLF (Nm)')
      | port_label('output', 4, 'ActSpdLF (rpm)')
      | port_label('output', 5, 'ActTempLF (C)')
      | port_label('output', 6, 'ActTqRF (Nm)')
      | port_label('output', 7, 'ActSpRF (rpm)')
      | port_label('output', 8, 'ActTempRF (C)')
      | port_label('output', 9, 'ActTqLR (Nm)')
      | port_label('output', 10, 'ActSpLR (rpm)')
      | port_label('output', 11, 'ActTempLR (C)')
      | port_label('output', 12, 'ActTqRR (Nm)')
      | port_label('output', 13, 'ActSpRR (rpm)')
      | port_label('output', 14, 'ActTempRR (Nm)')
      | port_label('output', 15, 'ActTqDeltaF (Nm)')
      | port_label('output', 16, 'ActSpDeltaF (rpm)')
      | port_label('output', 17, 'ActTqDeltaR (Nm)')
      | port_label('output', 18, 'ActSpDeltaR (rpm)')
      | port_label('output', 19, 'ActTqDeltaA (Nm')
      | port_label('output', 20, 'ActSqDeltaA (rpm)')
      | port_label('output', 21, 'ActTqTot (Nm)')
      | port_label('output', 22, 'ActSpAve (rpm)')
      | port_label('output', 23, 'ActPow (kW)')
      | port_label('output', 24, 'ActVehSp (kph)')
      | port_label('output', 25, 'TPTime (ms)')
      | port_label('output', 26, 'TPDistance (m)')
      | port_label('output', 27, 'FaultActive (bool)')
      | port_label('output', 28, 'WarningsActive (bool)')
      | port_label('output', 29, 'MeasuringStatus (bool)')
      | port_label('output', 30, 'SystemActive (bool)')
      | 
      | port_label('output', 31, 'UnitStatusLF (enum)')
      | port_label('output', 32, 'UnitStatusRF (enum)')
      | port_label('output', 33, 'UnitStatusLR (enum)')
      | port_label('output', 34, 'UnitStatusRR (enum)')
      | port_label('output', 35, 'WatchdogCnt (int)')
  Terminator{28..62} (35 alike) : Terminator
  wires:
  Ground1/1 -> RotoTestEthRXLogging/1(Cmd)
  RotoTestEthRXLogging/3(ActTqLF_Nm) -> Terminator36/1
  RotoTestEthRXLogging/29(MeasuringStatus) -> Terminator52/1
  RotoTestEthRXLogging/32(UnitsStatusRF) -> Terminator57/1
  RotoTestEthRXLogging/20(ActSpDeltaA_rpm) -> Terminator45/1
  RotoTestEthRXLogging/34(UnitsStatusRR) -> Terminator55/1
  RotoTestEthRXLogging/35(WatchdogCnt) -> Terminator62/1
  RotoTestEthRXLogging/27(FaultActive) -> Terminator60/1
  RotoTestEthRXLogging/28(WarningsActive) -> Terminator61/1
  RotoTestEthRXLogging/25(TPTime_ms) -> Terminator58/1
  RotoTestEthRXLogging/23(ActPow_kW) -> Terminator50/1
  RotoTestEthRXLogging/33(UnitsStatusLR) -> Terminator54/1
  RotoTestEthRXLogging/15(ActTqDeltaF_Nm) -> Terminator48/1
  RotoTestEthRXLogging/18(ActSpDeltaR_rpm) -> Terminator41/1
  RotoTestEthRXLogging/16(ActSpDeltaF_rpm) -> Terminator49/1
  RotoTestEthRXLogging/2(ProtocolVer) -> Terminator35/1
  RotoTestEthRXLogging/7(ActSpRF_rpm) -> Terminator32/1
  RotoTestEthRXLogging/17(ActTqDeltaR_Nm) -> Terminator40/1
  RotoTestEthRXLogging/21(ActTqTot_Nm) -> Terminator42/1
  RotoTestEthRXLogging/31(UnitsStatusLF) -> Terminator56/1
  RotoTestEthRXLogging/13(ActSpRR_rpm) -> Terminator46/1
  RotoTestEthRXLogging/22(ActSpAve_rpm) -> Terminator43/1
  RotoTestEthRXLogging/30(SystemActive) -> Terminator53/1
  RotoTestEthRXLogging/14(ActTempRR_Nm) -> Terminator47/1
  RotoTestEthRXLogging/1(ID) -> Terminator34/1
  RotoTestEthRXLogging/4(ActSpLF_rpm) -> Terminator37/1
  RotoTestEthRXLogging/6(ActTqRF_Nm) -> Terminator29/1
  RotoTestEthRXLogging/19(ActTqDeltaA_Nm) -> Terminator44/1
  RotoTestEthRXLogging/26(TPDistance_m) -> Terminator59/1
  RotoTestEthRXLogging/8(ActTempRF_C) -> Terminator33/1
  RotoTestEthRXLogging/10(ActSpLR_rpm) -> Terminator31/1
  RotoTestEthRXLogging/12(ActTqRR_Nm) -> Terminator39/1
  RotoTestEthRXLogging/5(ActTempLF_C) -> Terminator28/1
  RotoTestEthRXLogging/11(ActTempLR_C) -> Terminator38/1
  RotoTestEthRXLogging/9(ActTqLR_Nm) -> Terminator30/1
  RotoTestEthRXLogging/24(ActVehSp_kph) -> Terminator51/1

== system EV6_LUT_FourWheel_EV6Battery77p4kWh_PowerCorrected/Vehicle Under Test1/Vehicle/Rototest and ORNL Interface/To Rototest with Band-Aid/Mode Override ==
  Header : VSIGenLib/Header  not=''
  Mux6 : Mux
  SpTqLF : Constant  Value=0  OutDataTypeStr=uint8
  SpTqLR : Constant  Value=0  OutDataTypeStr=uint8
  SpTqRF : Constant  Value=0  OutDataTypeStr=uint8
  SpTqRR : Constant  Value=0  OutDataTypeStr=uint8
  Ovr : Outport
  wires:
  SpTqLF/1 -> Mux6/4
  SpTqRF/1 -> Mux6/3
  SpTqLR/1 -> Mux6/2
  SpTqRR/1 -> Mux6/1
  Mux6/1 -> Ovr/1

== system EV6_LUT_FourWheel_EV6Battery77p4kWh_PowerCorrected/Vehicle Under Test1/Vehicle/Rototest and ORNL Interface/To Rototest with Band-Aid/RotoTestEthTx ==
  RefLF_NmORrpm : Inport
  RefRF_NmORrpm : Inport  Port=2
  RefLR_NmORrpm : Inport  Port=3
  RefRR_NmORrpm : Inport  Port=4
  SpTqRR : Inport  Port=5
  SpTqLR : Inport  Port=6
  SpTqRF : Inport  Port=7
  SpTqLF : Inport  Port=8
  SystemActive : Inport  Port=9
  Constant : Constant  Value=255  OutDataTypeStr=uint8
  Constant1 : Constant  Value=0  OutDataTypeStr=uint8
  Constant2 : Constant  Value=0  OutDataTypeStr=uint8
  Constant3 : Constant  Value=0  OutDataTypeStr=uint8
  Defloater{,1..3} (4 alike) : VSIGenLib/Defloater  SystemSampleTime=-1  VariantActivationTime=update diagram  AllowFlexibleInterface=on  Latency=0  AutoFrameSizeCalculation=off
  Demux{,1..3} (4 alike) : Demux
  Header : VSIGenLib/Header  not=''
  ID1 : Constant  Value=hex2dec('D3')  OutDataTypeStr=uint8
  ID2 : Constant  Value=hex2dec('02')  OutDataTypeStr=uint8
  MATLAB Function : MATLAB Function  TreatAsAtomicUnit=on
  Mux : Mux  Inputs=25
  Packer : Subsystem
  ProtocolVer : Constant  Value=0  OutDataTypeStr=uint16
  SystemCtrlBits2 : Constant  Value=0  OutDataTypeStr=uint8
  Terminator : Terminator
  WatchdogCnt : simulink/Sources/Counter Free-Running  NumBits=8  tsamp=-1
  uint16 (unsigned 16) 2 : etargetslib/Byte Pack  datatypes={'uint16'}  byteAlign=1
  uint8 (unsigned 8) {1..9} (9 alike) : etargetslib/Byte Pack  datatypes={'uint8'}  byteAlign=1
  Output : Outport
  wires:
  uint8 (unsigned 8) 9/1 -> Mux/20
  Constant/1 -> uint8 (unsigned 8) 6/1
  Packer/1(SystemCtrlBits) -> Terminator/1
  SystemActive/1 -> Packer/5(SystemActive), MATLAB Function/5(SystemActive)
  SpTqLF/1 -> Packer/4(SpTqLF), MATLAB Function/4(SpTqLF)  "SpTqLF"
  SpTqRF/1 -> Packer/3(SpTqRF), MATLAB Function/3(SpTqRF)  "SpTqRF"
  SpTqLR/1 -> Packer/2(SpTqLR), MATLAB Function/2(SpTqLR)  "SpTqLR"
  SpTqRR/1 -> Packer/1(SpTqRR), MATLAB Function/1(SpTqRR)  "SpTqRR"
  RefLR_NmORrpm/1 -> Defloater2/1  "RefLR_NmORrpm"
  RefLF_NmORrpm/1 -> Defloater/1  "RefLF_NmORrpm"
  Demux3/2 -> Mux/17
  Constant3/1 -> uint8 (unsigned 8) 2/1  "Reserved23"
  Demux/2 -> Mux/5
  RefRR_NmORrpm/1 -> Defloater3/1  "RefRR_NmORrpm"
  uint8 (unsigned 8) 7/1 -> Mux/2
  SystemCtrlBits2/1 -> uint8 (unsigned 8) 5/1  "SystemCtrlBits2"
  Demux3/4 -> Mux/19
  Demux2/4 -> Mux/15
  uint8 (unsigned 8) 8/1 -> Mux/1
  Mux/1 -> Output/1  "bytesend"
  Demux/3 -> Mux/6
  Demux1/2 -> Mux/9
  MATLAB Function/1(y) -> uint8 (unsigned 8) 9/1  "Ref_Byte"
  Demux2/3 -> Mux/14
  Demux/4 -> Mux/7
  Demux2/1 -> Mux/12
  Defloater/1 -> Demux/1
  Defloater1/1 -> Demux1/1
  uint16 (unsigned 16) 2/1 -> Mux/3
  uint8 (unsigned 8) 1/1 -> Mux/22
  Demux2/2 -> Mux/13
  uint8 (unsigned 8) 3/1 -> Mux/24
  ProtocolVer/1 -> uint16 (unsigned 16) 2/1
  Demux1/1 -> Mux/8
  Demux3/1 -> Mux/16
  Demux/1 -> Mux/4
  uint8 (unsigned 8) 4/1 -> Mux/25
  ID1/1 -> uint8 (unsigned 8) 8/1
  Constant2/1 -> uint8 (unsigned 8) 3/1  "Reserved24"
  uint8 (unsigned 8) 2/1 -> Mux/23
  Demux1/3 -> Mux/10
  uint8 (unsigned 8) 5/1 -> Mux/21
  Demux3/3 -> Mux/18
  Defloater3/1 -> Demux3/1
  WatchdogCnt/1 -> uint8 (unsigned 8) 1/1  "WatchdogCnt"
  Constant1/1 -> uint8 (unsigned 8) 4/1  "Reserved25"
  Demux1/4 -> Mux/11
  RefRF_NmORrpm/1 -> Defloater1/1  "RefRF_NmORrpm"
  ID2/1 -> uint8 (unsigned 8) 7/1
  Defloater2/1 -> Demux2/1

== system EV6_LUT_FourWheel_EV6Battery77p4kWh_PowerCorrected/Vehicle Under Test1/Vehicle/Rototest and ORNL Interface/To Rototest with Band-Aid/TrqSpd Override ==
  Header : VSIGenLib/Header  not=''
  Mux2 : Mux
  RefLF_NmORrpm : Constant  Value=0
  RefLR_NmORrpm : Constant  Value=0
  RefRF_NmORrpm : Constant  Value=0
  RefRR_NmORrpm : Constant  Value=0
  Ovr : Outport
  wires:
  Mux2/1 -> Ovr/1
  RefRR_NmORrpm/1 -> Mux2/4
  RefLR_NmORrpm/1 -> Mux2/3
  RefLF_NmORrpm/1 -> Mux2/1
  RefRF_NmORrpm/1 -> Mux2/2

== system EV6_LUT_FourWheel_EV6Battery77p4kWh_PowerCorrected/Vehicle Under Test1/Vehicle/Vehicle Dynamics/Vehicle 14DOF/Brake Pressure ==
  BrkReq : Inport
  Bus Creator1 : BusCreator  Inputs=2
  Gain : Gain  Gain=BrakeMaxPrs
  Gain1 : Gain  Gain=0.4
  Gain2 : Gain  Gain=0.6
  Gain3 : Gain  Gain=0.5
  Gain4 : Gain  Gain=0.5
  Saturation{,1..3} (4 alike) : Saturate  UpperLimit=BrakeMaxPrs  LowerLimit=0  ZeroCross=off
  Scope : Scope
  Signal Specification : SignalSpecification  Unit=Pa
  Terminator : Terminator
  Vector Concatenate2 : Concatenate  NumInputs=4
  BrakePrs : Outport  Unit=Pa
  wires:
  Saturation3/1 -> Vector Concatenate2/4
  Saturation2/1 -> Vector Concatenate2/3
  Saturation1/1 -> Vector Concatenate2/2
  Saturation/1 -> Vector Concatenate2/1
  Vector Concatenate2/1 -> BrakePrs/1
  Gain4/1 -> Saturation3/1, Saturation2/1
  Gain3/1 -> Saturation1/1, Saturation/1
  Gain2/1 -> Gain3/1
  Gain1/1 -> Gain4/1
  Bus Creator1/1 -> Terminator/1  "WhlBrk"
  Signal Specification/1 -> Scope/1, Bus Creator1/2, Gain1/1, Gain2/1  "BrkPrs"
  Gain/1 -> Signal Specification/1
  BrkReq/1 -> Bus Creator1/1, Gain/1  "BrkReq"

== system EV6_LUT_FourWheel_EV6Battery77p4kWh_PowerCorrected/Vehicle Under Test1/Vehicle/Vehicle Dynamics/Vehicle 14DOF/Steering ==
  SteeringCmd : Inport
  Constant : Constant  Value=0
  Kinematic Steering : vehdynlibsteering/Kinematic Steering  StrgType=Parallel  StrgRatioType=Constant  Loc=Front  NrmlFctr=1  TrckWdth=1.9  WhlBase=ChassisDistCg2FrontAxle+ChassisDistCg2RearAxle  Db=0  StrgRng=2.91*pi  StrgAngBpts="[-6.2832   -5.0265   -3.7699   -2.5133   -1.2566         0    1.2566    2.5133    3.7699    5.0265    6.2832]"  StrgRatioTbl=|  StrgRatio=16.8  PctAckIn=off  PctAck=100  PctAckTbl=ones(1,11)*100  StrgArmLngth=0.1  RckCsLngth=0.5  TieRodLngth=0.248  D=0.2  PnnRadius=0.0057  PnnRadiusTbl="[0.0055    0.0055    0.0056    0.0057    0.0058    0.0057    0.0057    0.0057    0.0056    0.0055    0.0055]"  RodLngth=0.1  ParaArmLngth=0.9  aMode=2
      | [13.5000   13.3750   13.2500   13.1250   13.0000   13.0000   13.0000   13.1250   13.2500   13.3750   13.5000
      | ]
  Terminator1 : Terminator
  Vector Concatenate : Concatenate
  Vector Concatenate1 : Concatenate
  Vector Concatenate2 : Concatenate
  WhlAng : Outport  Unit=rad
  wires:
  SteeringCmd/1 -> Kinematic Steering/1
  Kinematic Steering/3 -> Vector Concatenate/2
  Constant/1 -> Vector Concatenate1/1, Vector Concatenate1/2
  Vector Concatenate/1 -> Vector Concatenate2/1  "FrontWheelAngles"
  Vector Concatenate1/1 -> Vector Concatenate2/2  "RearWheelAngles"
  Kinematic Steering/2 -> Vector Concatenate/1
  Vector Concatenate2/1 -> WhlAng/1
  Kinematic Steering/1 -> Terminator1/1

== system EV6_LUT_FourWheel_EV6Battery77p4kWh_PowerCorrected/Vehicle Under Test1/Vehicle/Vehicle Dynamics/Vehicle 14DOF/Subsystem1 ==
  Cgxyzdot : Inport
  CgXYZ : Inport  Port=2
  CgXYZdot : Inport  Port=3
  angles : Inport  Port=4
  pqr : Inport  Port=5
  Cgaxyz : Inport  Port=6
  Beta : Inport  Port=7
  GeomXYZ : Inport  Port=8
  GeomXYZdot : Inport  Port=9
  Cgxyzdotdot : Inport  Port=10
  Omega : Inport  Port=11
  Kappa : Inport  Port=12
  Alpha : Inport  Port=13
  XWheel : Inport  Port=14
  YWheel : Inport  Port=15
  dzWheel : Inport  Port=16
  Bus Creator1 : BusCreator  Inputs=29
  Bus Creator3 : BusCreator  Inputs=6
  Demux{,1..8} (9 alike) : Demux  Outputs=3
  Scope : Scope
  Subsystem : Subsystem
  Chassis : Outport  VectorParamsAs1DForOutWhenUnconnected=off
  Wheels : Outport  Port=2  VectorParamsAs1DForOutWhenUnconnected=off
  wires:
  Bus Creator1/1 -> Chassis/1  "Chassis"
  Omega/1 -> Bus Creator3/3  "Omega"
  dzWheel/1 -> Bus Creator3/6  "dZWheel"
  Kappa/1 -> Bus Creator3/1  "Kappa"
  Bus Creator3/1 -> Wheels/1  "Wheels"
  YWheel/1 -> Bus Creator3/5  "YWheel"
  XWheel/1 -> Bus Creator3/4  "XWheel"
  Alpha/1 -> Bus Creator3/2  "Alpha"
  Cgxyzdot/1 -> Subsystem/1(Cgxyzdot), Demux/1
  CgXYZ/1 -> Demux1/1
  CgXYZdot/1 -> Demux2/1
  angles/1 -> Subsystem/2(angles), Demux3/1
  pqr/1 -> Demux4/1
  Cgaxyz/1 -> Demux5/1
  GeomXYZdot/1 -> Demux7/1
  GeomXYZ/1 -> Demux6/1
  Demux/1 -> Bus Creator1/4  "xdot"
  Demux/2 -> Bus Creator1/5  "ydot"
  Demux/3 -> Bus Creator1/6  "zdot"
  Demux1/1 -> Bus Creator1/7  "X"
  Demux1/2 -> Bus Creator1/8  "Y"
  Demux1/3 -> Bus Creator1/9  "Z"
  Demux2/1 -> Bus Creator1/10  "Xdot"
  Demux2/2 -> Bus Creator1/11  "Ydot"
  Demux2/3 -> Bus Creator1/12  "Zdot"
  Demux3/1 -> Bus Creator1/13  "phi"
  Demux3/2 -> Bus Creator1/14  "theta"
  Demux3/3 -> Bus Creator1/15  "psi"
  Demux4/1 -> Bus Creator1/16  "p"
  Demux4/2 -> Bus Creator1/17  "q"
  Demux4/3 -> Bus Creator1/18  "r"
  Demux5/1 -> Bus Creator1/19  "ax"
  Demux5/2 -> Bus Creator1/20  "ay"
  Demux5/3 -> Bus Creator1/21  "az"
  Beta/1 -> Bus Creator1/22  "Beta"
  Demux6/1 -> Bus Creator1/23  "GeomX"
  Demux6/2 -> Bus Creator1/24  "GeomY"
  Demux6/3 -> Bus Creator1/25  "GeomZ"
  Demux7/1 -> Bus Creator1/26  "GeomXdot"
  Demux7/2 -> Bus Creator1/27  "GeomYdot"
  Demux7/3 -> Bus Creator1/28  "GeomZdot"
  Subsystem/1(VehSpd) -> Bus Creator1/29, Scope/1  "VehSpd"
  Cgxyzdotdot/1 -> Demux8/1
  Demux8/1 -> Bus Creator1/1  "xdotdot"
  Demux8/2 -> Bus Creator1/2  "ydotdot"
  Demux8/3 -> Bus Creator1/3  "zdotdot"

== system EV6_LUT_FourWheel_EV6Battery77p4kWh_PowerCorrected/Vehicle Under Test1/Vehicle/Vehicle Dynamics/Vehicle 14DOF/Subsystem4 ==
  Cgxyzdot : Inport
  CgXYZ : Inport  Port=2
  CgXYZdot : Inport  Port=3
  angles : Inport  Port=4
  pqr : Inport  Port=5
  Cgaxyz : Inport  Port=6
  Beta : Inport  Port=7
  GeomXYZ : Inport  Port=8
  GeomXYZdot : Inport  Port=9
  Omega : Inport  Port=10
  Kappa : Inport  Port=11
  Alpha : Inport  Port=12
  XWheel : Inport  Port=13
  YWheel : Inport  Port=14
  dzWheel : Inport  Port=15
  Bus Creator : BusCreator  Inputs=26
  Bus Creator3 : BusCreator  Inputs=6
  Demux{,1..7} (8 alike) : Demux  Outputs=3
  Subsystem : Subsystem
  Chassis : Outport  VectorParamsAs1DForOutWhenUnconnected=off
  Wheels : Outport  Port=2  VectorParamsAs1DForOutWhenUnconnected=off
  wires:
  Subsystem/1(VehSpd) -> Bus Creator/26  "VehSpd"
  Demux7/3 -> Bus Creator/25  "GeomZdot"
  Demux7/2 -> Bus Creator/24  "GeomYdot"
  Demux7/1 -> Bus Creator/23  "GeomXdot"
  Demux6/3 -> Bus Creator/22  "GeomZ"
  Demux6/2 -> Bus Creator/21  "GeomY"
  Demux6/1 -> Bus Creator/20  "GeomX"
  Beta/1 -> Bus Creator/19  "Beta"
  Demux5/3 -> Bus Creator/18  "az"
  Demux5/2 -> Bus Creator/17  "ay"
  Demux5/1 -> Bus Creator/16  "ax"
  Demux4/3 -> Bus Creator/15  "r"
  Demux4/2 -> Bus Creator/14  "q"
  Demux4/1 -> Bus Creator/13  "p"
  Demux3/3 -> Bus Creator/12  "psi"
  Demux3/2 -> Bus Creator/11  "theta"
  Demux3/1 -> Bus Creator/10  "phi"
  Demux2/3 -> Bus Creator/9  "Zdot"
  Demux2/2 -> Bus Creator/8  "Ydot"
  Demux2/1 -> Bus Creator/7  "Xdot"
  Demux1/3 -> Bus Creator/6  "Z"
  Demux1/2 -> Bus Creator/5  "Y"
  Demux1/1 -> Bus Creator/4  "X"
  Demux/3 -> Bus Creator/3  "zdot"
  Demux/2 -> Bus Creator/2  "ydot"
  Demux/1 -> Bus Creator/1  "xdot"
  GeomXYZ/1 -> Demux6/1
  GeomXYZdot/1 -> Demux7/1
  Cgaxyz/1 -> Demux5/1
  pqr/1 -> Demux4/1
  angles/1 -> Demux3/1, Subsystem/2(angles)
  CgXYZdot/1 -> Demux2/1
  CgXYZ/1 -> Demux1/1
  Cgxyzdot/1 -> Demux/1, Subsystem/1(Cgxyzdot)
  Alpha/1 -> Bus Creator3/2  "Alpha"
  XWheel/1 -> Bus Creator3/4  "XWheel"
  YWheel/1 -> Bus Creator3/5  "YWheel"
  Bus Creator3/1 -> Wheels/1  "Wheels"
  Kappa/1 -> Bus Creator3/1  "Kappa"
  dzWheel/1 -> Bus Creator3/6  "dZWheel"
  Omega/1 -> Bus Creator3/3  "Omega"
  Bus Creator/1 -> Chassis/1  "Chassis"
